simulink model "Tractor_HIT_Discrete"  (R2024a)
settings: Solver=ode1  StartTime=0.0  StopTime=60  FixedStep=0.001  RelTol=1e-3
values from neighbouring files (symbols this model uses):
  ANRtarget = 1.05    [Engine1204.sldd]    (also in Engine1204_init_r1.m; Engine2004.sldd; Engine2004_init.m; Engine3204.sldd)
  BackPrs = 3.0 4.2 5.5 7.0 8.5 10.0 11.5 12.5    [Engine1204.sldd]    (also in Engine1204_init_r1.m = [3.0, 4.2, 5.5, 7.0, 8.5, 10.0, 11.5, 12.5]; Engine2004.sldd = 3.0 4.2 5.5 7.0 8.5 10.0 11.5 12.5 13.5 14.5 15.0 15.5 16.0 ; Engine2004_init.m = [3.0,4.2,5.5,7.0,8.5,10.0,11.5,12.5,13.5,14.5,15.0,15.5,16.0; Engine3204.sldd = 3.0 4.5 6.0 7.5 9.0 10.5 12.0 13.0 13.8 14.4 14.8 15.2 15.6 )
  BackPrs_x = 50.0 100.0 150.0 200.0 250.0 300.0 350.0 400.0    [Engine1204.sldd]    (also in Engine1204_init_r1.m = [50:50:400]; Engine2004.sldd = 50.0 100.0 150.0 200.0 250.0 300.0 350.0 400.0 450.0 500.0 5; Engine2004_init.m = [50:50:800]; Engine3204.sldd = 100.0 200.0 300.0 400.0 500.0 600.0 700.0 800.0 900.0 1000.0)
  Bf = 0.38    [Engine1204.sldd]    (also in Engine2004.sldd; Engine3204.sldd)
  Br = 0.47    [Engine1204.sldd]    (also in Engine2004.sldd; Engine3204.sldd)
  BSFC = 320.0 285.0 275.0 280.0 290.0 300.0 310.0 260.0 225.0 215.0 220.0 228.0 240.0 250.0 235.0 208.0 202.0 205.0 212.0 222.0 232.0 230.0 205.0 200.0 204.0 210.0 220.0 230.0 232.0 207.0 203.0 206.0 213.0 224.0 235.0    [Engine1204.sldd]    (also in Engine1204_init_r1.m = [320,285,275,280,290,300,310; Engine2004.sldd = 315.0 280.0 270.0 275.0 285.0 295.0 305.0 255.0 220.0 210.0 ; Engine2004_init.m = [315,280,270,275,285,295,305; Engine3204.sldd = 310.0 275.0 265.0 270.0 280.0 290.0 300.0 250.0 215.0 205.0 )
  BSFC_x = 700.0 1200.0 1400.0 1600.0 1800.0 2000.0 2200.0    [Engine1204.sldd]    (also in Engine1204_init_r1.m = [700,1200,1400,1600,1800,2000,2200]; Engine2004.sldd = 800.0 1200.0 1400.0 1600.0 1800.0 2000.0 2200.0; Engine2004_init.m = [800,1200,1400,1600,1800,2000,2200]; Engine3204.sldd = 800.0 1000.0 1200.0 1400.0 1600.0 1800.0 2100.0)
  BSFC_y = 12.0 24.0 36.0 48.0 54.0    [Engine1204.sldd]    (also in Engine1204_init_r1.m = [12,24,36,48,54]; Engine2004.sldd = 20.0 40.0 60.0 80.0 100.0; Engine2004_init.m = [20,40,60,80,100]; Engine3204.sldd = 30.0 60.0 90.0 120.0 150.0)
  CO = 2.4 1.7 1.5 1.6 1.8 2.1 2.7 1.1 0.72 0.65 0.68 0.78 0.92 1.3 0.7 0.55 0.5 0.53 0.6 0.72 0.95 1.2 0.9 0.85 0.88 0.96 1.1 1.45 3.2 2.3 2.1 2.25 2.5 2.85 3.8    [Engine1204.sldd]    (also in Engine1204_init_r1.m = [; Engine2004.sldd = 2.3 1.63 1.44 1.54 1.73 2.02 2.56 1.05 0.68 0.61 0.64 0.74 0; Engine2004_init.m = [; Engine3204.sldd = 2.2 1.56 1.38 1.48 1.66 1.94 2.46 1.0 0.65 0.58 0.61 0.7 0.8)
  CO_x = 700.0 1200.0 1400.0 1600.0 1800.0 2000.0 2200.0    [Engine1204.sldd]    (also in Engine1204_init_r1.m = [700,1200,1400,1600,1800,2000,2200]; Engine2004.sldd = 800.0 1200.0 1400.0 1600.0 1800.0 2000.0 2200.0; Engine2004_init.m = [800,1200,1400,1600,1800,2000,2200]; Engine3204.sldd = 800.0 1000.0 1200.0 1400.0 1600.0 1800.0 2100.0)
  CO_y = 12.0 24.0 36.0 48.0 54.0    [Engine1204.sldd]    (also in Engine1204_init_r1.m = [12,24,36,48,54]; Engine2004.sldd = 20.0 40.0 60.0 80.0 100.0; Engine2004_init.m = [20,40,60,80,100]; Engine3204.sldd = 30.0 60.0 90.0 120.0 150.0)
  Df = 1.4    [Engine1204.sldd]    (also in Engine2004.sldd; Engine3204.sldd)
  dfmax = 0.1    [Engine1204.sldd]    (also in Engine2004.sldd; Engine3204.sldd)
  dfmin = 0.035    [Engine1204.sldd]    (also in Engine2004.sldd; Engine3204.sldd)
  DOCdPrs = 0.2 0.5 0.8 1.1 1.2    [Engine1204.sldd]    (also in Engine1204_init_r1.m = [0.2  0.5  0.8  1.1  1.2]; Engine2004.sldd = 0.25 0.55 0.85 1.15 1.3; Engine2004_init.m = [0.25,0.55,0.85,1.15,1.30]; Engine3204.sldd = 0.25 0.55 0.85 1.15 1.3 1.45)
  DOCdPrs_x = 50.0 150.0 250.0 350.0 400.0    [Engine1204.sldd]    (also in Engine1204_init_r1.m = [50  150  250  350  400]; Engine2004.sldd = 100.0 250.0 400.0 600.0 800.0; Engine2004_init.m = [100 250 400 600 800]; Engine3204.sldd = 100.0 250.0 400.0 600.0 800.0 1200.0)
  DPFdPrs = 0.3 0.5 0.7 0.9 0.6 1.0 1.4 1.8 0.9 1.5 2.1 2.6 1.2 2.0 2.7 2.8    [Engine1204.sldd]    (also in Engine1204_init_r1.m = [0.3  0.5  0.7  0.9; Engine2004.sldd = 0.35 0.6 0.85 1.1 0.7 1.15 1.6 2.0 1.05 1.7 2.3 2.5 1.4 2.2 ; Engine2004_init.m = [0.35,0.60,0.85,1.10; Engine3204.sldd = 0.35 0.7 1.05 1.4 1.7 2.0 2.2 2.4 2.55 2.65 2.7 2.75 0.6 1.1)
  DPFdPrs_x = 100.0 200.0 300.0 400.0    [Engine1204.sldd]    (also in Engine1204_init_r1.m = [100: 100 : 400]; Engine2004.sldd = 100.0 300.0 500.0 700.0; Engine2004_init.m = [100:200:700]; Engine3204.sldd = 100.0 200.0 300.0 400.0 500.0 600.0 700.0 800.0 900.0 1000.0)
  DPFdPrs_y = 0.0 6.0 12.0 20.0    [Engine1204.sldd]    (also in Engine1204_init_r1.m = [0 6 12 20 ]; Engine2004.sldd = 0.0 8.0 16.0 24.0; Engine2004_init.m = [0 8 16 24]; Engine3204.sldd = 0.0 10.0 20.0 30.0)
  DPFSootBurn = 0.0 0.0 0.0 0.0 0.0 0.2 0.4 0.6 0.8 1.0 1.2 2.4 3.6 4.8 6.0 6.0 12.0 18.0 24.0 30.0 12.0 24.0 36.0 48.0 60.0 20.0 40.0 60.0 80.0 100.0 22.0 44.0 66.0 88.0 110.0    [Engine1204.sldd]    (also in Engine1204_init_r1.m = [0,0,0,0,0; Engine2004.sldd = 0.0 0.0 0.0 0.0 0.0 0.5 1.0 1.5 2.0 2.5 3.0 6.0 9.0 12.0 15.; Engine2004_init.m = [0,0,0,0,0; Engine3204.sldd = 0.0 0.0 0.0 0.0 0.0 0.5 1.0 1.5 2.0 2.5 3.0 6.0 9.0 12.0 15.)
  DPFSootBurn_x = 100.0 200.0 300.0 400.0 500.0    [Engine1204.sldd]    (also in Engine1204_init_r1.m = [100,200,300,400,500]; Engine2004.sldd = 200.0 300.0 400.0 500.0 650.0; Engine2004_init.m = [200,300,400,500,650]; Engine3204.sldd = 200.0 300.0 400.0 500.0 650.0)
  DPFSootBurn_y = 400.0 450.0 500.0 550.0 600.0 650.0 680.0    [Engine1204.sldd]    (also in Engine1204_init_r1.m = [400,450,500,550,600,650,680]; Engine2004.sldd; Engine2004_init.m = [400,450,500,550,600,650,680]; Engine3204.sldd)
  Dr = 1.8    [Engine1204.sldd]    (also in Engine2004.sldd; Engine3204.sldd)
  drmax = 0.12    [Engine1204.sldd]    (also in Engine2004.sldd; Engine3204.sldd)
  drmin = 0.04    [Engine1204.sldd]    (also in Engine2004.sldd; Engine3204.sldd)
  EGRKi = 0.03    [Engine1204.sldd]    (also in Engine1204_init_r1.m; Engine2004.sldd; Engine2004_init.m; Engine3204.sldd)
  EGRKp = 3.5999999999999996    [Engine1204.sldd]    (also in Engine1204_init_r1.m = 3.6; Engine2004.sldd; Engine2004_init.m = 3.6; Engine3204.sldd)
  EGRMax = 1.0    [Engine1204.sldd]    (also in Engine1204_init_r1.m = 1; Engine2004.sldd; Engine2004_init.m = 1; Engine3204.sldd)
  EGRMin = 0.0    [Engine1204.sldd]    (also in Engine1204_init_r1.m = 0; Engine2004.sldd; Engine2004_init.m = 0; Engine3204.sldd)
  EGRRatio = 0.0 0.0 0.0 0.0 0.0 0.0 0.0 0.0 0.04 0.03 0.03 0.02 0.02 0.01 0.0 0.08 0.07 0.06 0.05 0.04 0.03 0.0 0.13 0.12 0.11 0.1 0.09 0.08 0.0 0.18 0.17 0.16 0.15 0.14 0.13 0.0 0.22 0.21 0.2 0.19 0.18 0.17    [Engine1204.sldd]    (also in Engine1204_init_r1.m = [; Engine2004.sldd; Engine2004_init.m = [; Engine3204.sldd)
  EGRRatio_x = 700.0 1200.0 1400.0 1600.0 1800.0 2000.0 2200.0    [Engine1204.sldd]    (also in Engine1204_init_r1.m = [700,1200,1400,1600,1800,2000,2200]; Engine2004.sldd = 800.0 1200.0 1400.0 1600.0 1800.0 2000.0 2200.0; Engine2004_init.m = [800,1200,1400,1600,1800,2000,2200]; Engine3204.sldd = 800.0 1000.0 1200.0 1400.0 1600.0 1800.0 2100.0)
  EGRRatio_y = 0.0 20.0 40.0 60.0 80.0 100.0    [Engine1204.sldd]    (also in Engine1204_init_r1.m = [0,20,40,60,80,100]; Engine2004.sldd; Engine2004_init.m = [0,20,40,60,80,100]; Engine3204.sldd)
  EGRTgt = 0.25 0.22 0.2 0.18 0.16 0.12 0.1 0.2 0.18 0.15 0.14 0.12 0.1 0.08 0.12 0.13 0.1 0.09 0.08 0.06 0.04 0.08 0.09 0.07 0.06 0.05 0.03 0.02 0.05 0.06 0.04 0.03 0.02 0.01 0.0    [Engine1204.sldd]    (also in Engine1204_init_r1.m = [0.25,0.22,0.20,0.18,0.16,0.12,0.10; Engine2004.sldd = 0.24 0.21 0.19 0.17 0.15 0.11 0.09 0.19 0.17 0.14 0.13 0.11 ; Engine2004_init.m = [0.24,0.21,0.19,0.17,0.15,0.11,0.09; Engine3204.sldd = 0.23 0.2 0.18 0.16 0.14 0.1 0.08 0.18 0.16 0.13 0.12 0.1 0.0)
  EGRTgt_x = 700.0 1200.0 1400.0 1600.0 1800.0 2000.0 2200.0    [Engine1204.sldd]    (also in Engine1204_init_r1.m = [700,1200,1400,1600,1800,2000,2200]; Engine2004.sldd = 800.0 1200.0 1400.0 1600.0 1800.0 2000.0 2200.0; Engine2004_init.m = [800,1200,1400,1600,1800,2000,2200]; Engine3204.sldd = 800.0 1000.0 1200.0 1400.0 1600.0 1800.0 2100.0)
  EGRTgt_y = 12.0 24.0 36.0 48.0 54.0    [Engine1204.sldd]    (also in Engine1204_init_r1.m = [12,24,36,48,54]; Engine2004.sldd = 20.0 40.0 60.0 80.0 100.0; Engine2004_init.m = [20,40,60,80,100]; Engine3204.sldd = 30.0 60.0 90.0 120.0 150.0)
  EGT = 197.0 257.0 287.0 297.0 287.0 267.0 247.0 267.0 357.0 397.0 407.0 392.0 367.0 347.0 337.0 437.0 472.0 482.0 462.0 437.0 407.0 367.0 477.0 502.0 512.0 492.0 467.0 437.0 377.0 487.0 510.0 520.0 500.0 477.0 447.0    [Engine1204.sldd]    (also in Engine1204_init_r1.m = [470,530,560,570,560,540,520; Engine2004.sldd = 187.0 247.0 277.0 287.0 277.0 257.0 237.0 257.0 347.0 387.0 ; Engine2004_init.m = [460,520,550,560,550,530,510; Engine3204.sldd = 307.0 327.0 338.0 327.0 307.0 277.0 237.0 322.0 337.0 332.0 )
  EGT_x = 700.0 1200.0 1400.0 1600.0 1800.0 2000.0 2200.0    [Engine1204.sldd]    (also in Engine1204_init_r1.m = [700,1200,1400,1600,1800,2000,2200]; Engine2004.sldd = 800.0 1200.0 1400.0 1600.0 1800.0 2000.0 2200.0; Engine2004_init.m = [800,1200,1400,1600,1800,2000,2200]; Engine3204.sldd = 800.0 1000.0 1200.0 1400.0 1600.0 1800.0 2100.0)
  EGT_y = 12.0 24.0 36.0 48.0 54.0    [Engine1204.sldd]    (also in Engine1204_init_r1.m = [12,24,36,48,54]; Engine2004.sldd = 20.0 40.0 60.0 80.0 100.0; Engine2004_init.m = [20,40,60,80,100]; Engine3204.sldd = 30.0 60.0 90.0 120.0 150.0)
  EngCsup = 0.35594 0.35501499999999997 0.353535 0.35242500000000004 0.351685 0.35150000000000003 0.35187 0.352795 0.35446 0.356865    [Engine1204.sldd]    (also in Engine2004.sldd; Engine3204.sldd)
  EngineSpdTgt = 700.0 850.0 1000.0 1150.0 1300.0 1450.0 1600.0 1750.0 1900.0 2050.0 2200.0    [Engine1204.sldd]    (also in Engine1204_init_r1.m = [700:150:2200]; Engine2004.sldd; Engine2004_init.m = [700:150:2200]; Engine3204.sldd = 800.0 930.0 1060.0 1190.0 1320.0 1450.0 1580.0 1710.0 1840.0)
  EngineSpdTgt_x = 0.0 10.0 20.0 30.0 40.0 50.0 60.0 70.0 80.0 90.0 100.0    [Engine1204.sldd]    (also in Engine1204_init_r1.m = [0:10:100]; Engine2004.sldd; Engine2004_init.m = [0:10:100]; Engine3204.sldd)
  EngineTrq = 70.0 110.0 130.0 125.0 115.0 100.0 85.0 180.0 280.0 320.0 310.0 285.0 250.0 220.0 260.0 370.0 410.0 395.0 365.0 320.0 280.0 300.0 420.0 450.0 435.0 400.0 350.0 300.0 310.0 435.0 460.0 445.0 410.0 355.0 305.0    [Engine1204.sldd]    (also in Engine1204_init_r1.m = [70,110,130,125,115,100,85; Engine2004.sldd = 130.0 200.0 240.0 230.0 210.0 180.0 150.0 320.0 480.0 550.0 ; Engine2004_init.m = [130,200,240,230,210,180,150; Engine3204.sldd = 210.0 320.0 380.0 360.0 330.0 290.0 240.0 510.0 760.0 870.0 )
  EngineTrq_x = 700.0 1200.0 1400.0 1600.0 1800.0 2000.0 2200.0    [Engine1204.sldd]    (also in Engine1204_init_r1.m = [700,1200,1400,1600,1800,2000,2200]; Engine2004.sldd = 800.0 1200.0 1400.0 1600.0 1800.0 2000.0 2200.0; Engine2004_init.m = [800,1200,1400,1600,1800,2000,2200]; Engine3204.sldd = 800.0 1000.0 1200.0 1400.0 1600.0 1800.0 2100.0)
  EngineTrq_y = 12.0 24.0 36.0 48.0 54.0    [Engine1204.sldd]    (also in Engine1204_init_r1.m = [12,24,36,48,54]; Engine2004.sldd = 20.0 40.0 60.0 80.0 100.0; Engine2004_init.m = [20,40,60,80,100]; Engine3204.sldd = 30.0 60.0 90.0 120.0 150.0)
  EngSpd = 800.0 1000.0 1200.0 1400.0 1600.0 1800.0 2000.0 2200.0 2400.0 2600.0    [Engine1204.sldd]    (also in Engine2004.sldd; Engine3204.sldd)
  EngTrq = 667.0 700.0 768.0 830.0 885.0 860.0 789.0 690.0 542.0 352.0    [Engine1204.sldd]    (also in Engine2004.sldd; Engine3204.sldd)
  etaCO = 0.0 0.0 0.0 0.0 0.6 0.45 0.3 0.15 0.92 0.85 0.75 0.6 0.98 0.95 0.9 0.82 0.99 0.97 0.94 0.88    [Engine1204.sldd]    (also in Engine1204_init_r1.m = [0.00	0.00	0.00	0.00; Engine2004.sldd; Engine2004_init.m = [0.00	0.00	0.00	0.00; Engine3204.sldd)
  etaCO_x = 10000.0 25000.0 40000.0 60000.0    [Engine1204.sldd]    (also in Engine1204_init_r1.m = [10000  25000  40000  60000]; Engine2004.sldd; Engine2004_init.m = [10000 25000 40000 60000]; Engine3204.sldd)
  etaCO_y = 120.0 200.0 280.0 360.0 450.0    [Engine1204.sldd]    (also in Engine1204_init_r1.m = [120, 200, 280, 360, 450]; Engine2004.sldd; Engine2004_init.m = [120,200,280,360,450]; Engine3204.sldd)
  etaHC = 0.0 0.0 0.0 0.0 0.5 0.35 0.2 0.1 0.88 0.8 0.68 0.5 0.96 0.92 0.86 0.75 0.98 0.95 0.91 0.83    [Engine1204.sldd]    (also in Engine1204_init_r1.m = [0.00	0.00	0.00	0.00; Engine2004.sldd; Engine2004_init.m = [0.00	0.00	0.00	0.00; Engine3204.sldd)
  etaHC_x = 10000.0 25000.0 40000.0 60000.0    [Engine1204.sldd]    (also in Engine1204_init_r1.m = [10000  25000  40000  60000]; Engine2004.sldd; Engine2004_init.m = [10000 25000 40000 60000]; Engine3204.sldd)
  etaHC_y = 120.0 200.0 280.0 360.0 450.0    [Engine1204.sldd]    (also in Engine1204_init_r1.m = [120, 200, 280, 360, 450]; Engine2004.sldd; Engine2004_init.m = [120,200,280,360,450]; Engine3204.sldd)
  etaNO2 = 0.0 0.0 0.0 0.0 0.2 0.15 0.1 0.05 0.4 0.33 0.25 0.18 0.55 0.48 0.4 0.3 0.6 0.53 0.45 0.35    [Engine1204.sldd]    (also in Engine1204_init_r1.m = [0.00	0.00	0.00	0.00; Engine2004.sldd; Engine2004_init.m = [0.00	0.00	0.00	0.00; Engine3204.sldd)
  etaNO2_x = 10000.0 25000.0 40000.0 60000.0    [Engine1204.sldd]    (also in Engine1204_init_r1.m = [10000  25000  40000  60000]; Engine2004.sldd; Engine2004_init.m = [10000 25000 40000 60000]; Engine3204.sldd)
  etaNO2_y = 120.0 200.0 280.0 360.0 450.0    [Engine1204.sldd]    (also in Engine1204_init_r1.m = [120, 200, 280, 360, 450]; Engine2004.sldd; Engine2004_init.m = [120,200,280,360,450]; Engine3204.sldd)
  etaPM = 0.995 0.992 0.988 0.98 0.996 0.994 0.99 0.985 0.997 0.995 0.992 0.988    [Engine1204.sldd]    (also in Engine1204_init_r1.m = [0.995  0.992  0.988  0.980; Engine2004.sldd; Engine2004_init.m = [0.995  0.992  0.988  0.980; Engine3204.sldd)
  etaPM_x = 10000.0 25000.0 40000.0 60000.0    [Engine1204.sldd]    (also in Engine1204_init_r1.m = [10000  25000  40000  60000]; Engine2004.sldd; Engine2004_init.m = [10000 25000 40000 60000]; Engine3204.sldd)
  etaPM_y = 150.0 300.0 450.0    [Engine1204.sldd]    (also in Engine1204_init_r1.m = [150, 300, 450]; Engine2004.sldd; Engine2004_init.m = [150,300,450]; Engine3204.sldd)
  FuelCyleMax = 40.0 45.0 50.0 52.0 54.0 50.0 60.0 65.0 66.0 68.0 52.0 64.0 66.0 67.0 68.0 50.0 62.0 64.0 65.0 66.0 48.0 58.0 60.0 61.0 62.0 42.0 50.0 52.0 53.0 54.0 38.0 44.0 46.0 47.0 48.0    [Engine1204.sldd]    (also in Engine1204_init_r1.m = [40,45,50,52,54; Engine2004.sldd = 65.0 75.0 82.0 88.0 92.0 75.0 88.0 94.0 98.0 102.0 78.0 92.0; Engine2004_init.m = [65,75,82,88,92; Engine3204.sldd = 95.0 110.0 125.0 140.0 155.0 110.0 130.0 145.0 160.0 175.0 1)
  FuelCyleMax_x = 80.0 140.0 200.0 260.0 320.0    [Engine1204.sldd]    (also in Engine1204_init_r1.m = [80,140,200,260,320]; Engine2004.sldd = 150.0 300.0 450.0 600.0 750.0; Engine2004_init.m = [150,300,450,600,750]; Engine3204.sldd = 250.0 500.0 750.0 1000.0 1300.0)
  FuelCyleMax_y = 700.0 1200.0 1400.0 1600.0 1800.0 2000.0 2200.0    [Engine1204.sldd]    (also in Engine1204_init_r1.m = [700,1200,1400,1600,1800,2000,2200]; Engine2004.sldd = 800.0 1200.0 1400.0 1600.0 1800.0 2000.0 2200.0; Engine2004_init.m = [800,1200,1400,1600,1800,2000,2200]; Engine3204.sldd = 800.0 1000.0 1200.0 1400.0 1600.0 1800.0 2100.0)
  FuelCyleMaxSw = 0.0    [Engine1204.sldd]    (also in Engine1204_init_r1.m = 0; Engine2004.sldd; Engine2004_init.m = 0; Engine3204.sldd)
  FuelCyleMin = 10.0    [Engine1204.sldd]    (also in Engine1204_init_r1.m = 10; Engine2004.sldd = 12.0; Engine2004_init.m = 12; Engine3204.sldd = 15.0)
  FuelKd = 0.0    [Engine1204.sldd]    (also in Engine1204_init_r1.m = 0; Engine2004.sldd; Engine2004_init.m = 0; Engine3204.sldd)
  FuelKi = 0.0162    [Engine1204.sldd]    (also in Engine1204_init_r1.m; Engine2004.sldd = 0.0198; Engine2004_init.m = 0.0198; Engine3204.sldd = 0.025199999999999997)
  FuelKp = 0.054    [Engine1204.sldd]    (also in Engine1204_init_r1.m; Engine2004.sldd = 0.066; Engine2004_init.m = 0.066; Engine3204.sldd = 0.083999999999999991)
  g = 9.81    [Engine1204.sldd]    (also in Engine2004.sldd; Engine3204.sldd)
  GearA = -2.9 0.0 6.0 2.5 1.0    [Engine1204.sldd]    (also in Engine2004.sldd; Engine3204.sldd)
  GearAC = -1.0 0.0 1.0 2.0 3.0    [Engine1204.sldd]    (also in Engine2004.sldd; Engine3204.sldd)
  GearFront = 17.574    [Engine1204.sldd]    (also in Engine2004.sldd; Engine3204.sldd)
  GearM = 2.33 1.75 1.4 1.0    [Engine1204.sldd]    (also in Engine2004.sldd; Engine3204.sldd)
  GearMC = 1.0 2.0 3.0 4.0    [Engine1204.sldd]    (also in Engine2004.sldd; Engine3204.sldd)
  GearRef = 14.6    [Engine1204.sldd]    (also in Engine2004.sldd; Engine3204.sldd)
  HC = 0.85 0.6 0.52 0.55 0.62 0.7 0.9 0.4 0.22 0.2 0.21 0.26 0.32 0.48 0.25 0.18 0.17 0.18 0.21 0.26 0.36 0.32 0.24 0.23 0.25 0.28 0.33 0.42 0.55 0.42 0.4 0.43 0.48 0.54 0.68    [Engine1204.sldd]    (also in Engine1204_init_r1.m = [; Engine2004.sldd = 0.82 0.58 0.5 0.53 0.6 0.68 0.87 0.38 0.21 0.19 0.2 0.24 0.3; Engine2004_init.m = [; Engine3204.sldd = 0.8 0.56 0.48 0.51 0.58 0.66 0.84 0.37 0.2 0.18 0.19 0.23 0.)
  HC_x = 700.0 1200.0 1400.0 1600.0 1800.0 2000.0 2200.0    [Engine1204.sldd]    (also in Engine1204_init_r1.m = [700,1200,1400,1600,1800,2000,2200]; Engine2004.sldd = 800.0 1200.0 1400.0 1600.0 1800.0 2000.0 2200.0; Engine2004_init.m = [800,1200,1400,1600,1800,2000,2200]; Engine3204.sldd = 800.0 1000.0 1200.0 1400.0 1600.0 1800.0 2100.0)
  HC_y = 12.0 24.0 36.0 48.0 54.0    [Engine1204.sldd]    (also in Engine1204_init_r1.m = [12,24,36,48,54]; Engine2004.sldd = 20.0 40.0 60.0 80.0 100.0; Engine2004_init.m = [20,40,60,80,100]; Engine3204.sldd = 30.0 60.0 90.0 120.0 150.0)
  hf = 0.35    [Engine1204.sldd]    (also in Engine2004.sldd; Engine3204.sldd)
  hr = 0.4    [Engine1204.sldd]    (also in Engine2004.sldd; Engine3204.sldd)
  IdleEngSpd = 700.0    [Engine1204.sldd]    (also in Engine2004.sldd; Engine3204.sldd)
  IdleThrottle = 0.3    [Engine1204.sldd]    (also in Engine2004.sldd; Engine3204.sldd)
  Inertia = 0.9    [Engine1204.sldd]    (also in Engine1204_init_r1.m; Engine2004.sldd = 1.4; Engine2004_init.m = 1.4; Engine3204.sldd = 2.0)
  Intake = 80.0 140.0 160.0 180.0 190.0 195.0 200.0 130.0 210.0 240.0 260.0 270.0 275.0 280.0 170.0 270.0 310.0 330.0 340.0 345.0 350.0 190.0 320.0 360.0 380.0 390.0 395.0 400.0 200.0 340.0 380.0 400.0 410.0 415.0 420.0    [Engine1204.sldd]    (also in Engine1204_init_r1.m = [80,140,160,180,190,195,200; Engine2004.sldd = 160.0 240.0 280.0 310.0 330.0 340.0 350.0 250.0 380.0 440.0 ; Engine2004_init.m = [160,240,280,310,330,340,350; Engine3204.sldd = 280.0 420.0 490.0 540.0 570.0 585.0 600.0 430.0 660.0 760.0 )
  Intake_x = 700.0 1200.0 1400.0 1600.0 1800.0 2000.0 2200.0    [Engine1204.sldd]    (also in Engine1204_init_r1.m = [700,1200,1400,1600,1800,2000,2200]; Engine2004.sldd = 800.0 1200.0 1400.0 1600.0 1800.0 2000.0 2200.0; Engine2004_init.m = [800,1200,1400,1600,1800,2000,2200]; Engine3204.sldd = 800.0 1000.0 1200.0 1400.0 1600.0 1800.0 2100.0)
  Intake_y = 12.0 24.0 36.0 48.0 54.0    [Engine1204.sldd]    (also in Engine1204_init_r1.m = [12,24,36,48,54]; Engine2004.sldd = 20.0 40.0 60.0 80.0 100.0; Engine2004_init.m = [20,40,60,80,100]; Engine3204.sldd = 30.0 60.0 90.0 120.0 150.0)
  IntakePrs = 1.0 1.1 1.22 1.35 1.48 1.6 1.7 1.0 1.12 1.24 1.37 1.5 1.62 1.72 1.0 1.13 1.25 1.38 1.51 1.63 1.73 1.0 1.14 1.26 1.39 1.52 1.64 1.74 1.0 1.15 1.27 1.4 1.53 1.65 1.75 1.0 1.16 1.28 1.41 1.54 1.66 1.76    [Engine1204.sldd]    (also in Engine1204_init_r1.m = [; Engine2004.sldd = 1.0 1.11 1.23 1.36 1.49 1.61 1.71 1.0 1.13 1.25 1.38 1.51 1.; Engine2004_init.m = [; Engine3204.sldd = 1.0 1.12 1.24 1.37 1.5 1.62 1.72 1.0 1.14 1.26 1.39 1.52 1.6)
  IntakePrs_x = 700.0 1200.0 1400.0 1600.0 1800.0 2000.0 2200.0    [Engine1204.sldd]    (also in Engine1204_init_r1.m = [700,1200,1400,1600,1800,2000,2200]; Engine2004.sldd = 800.0 1200.0 1400.0 1600.0 1800.0 2000.0 2200.0; Engine2004_init.m = [800,1200,1400,1600,1800,2000,2200]; Engine3204.sldd = 800.0 1000.0 1200.0 1400.0 1600.0 1800.0 2100.0)
  IntakePrs_y = 0.0 20.0 40.0 60.0 80.0 100.0    [Engine1204.sldd]    (also in Engine1204_init_r1.m = [0,20,40,60,80,100]; Engine2004.sldd; Engine2004_init.m = [0,20,40,60,80,100]; Engine3204.sldd)
  IntakePrsInit = 1.35    [Engine1204.sldd]    (also in Engine1204_init_r1.m; Engine2004.sldd; Engine2004_init.m; Engine3204.sldd)
  IntakeSw = 0    [Engine1204.sldd]    (also in Engine1204_init_r1.m = false; Engine2004.sldd; Engine2004_init.m = false; Engine3204.sldd)
  IntakeTC = 0.1    [Engine1204.sldd]    (also in Engine1204_init_r1.m; Engine2004.sldd; Engine2004_init.m; Engine3204.sldd)
  IntakeTemp = 25.0 28.0 30.0 32.0 34.0 36.0 38.0 25.0 38.0 40.0 42.0 44.0 46.0 48.0 25.0 48.0 50.0 52.0 54.0 56.0 58.0 25.0 58.0 60.0 62.0 64.0 66.0 68.0 25.0 66.0 68.0 70.0 72.0 74.0 76.0 25.0 72.0 74.0 76.0 78.0 80.0 82.0    [Engine1204.sldd]    (also in Engine1204_init_r1.m = [; Engine2004.sldd = 25.0 29.0 31.0 33.0 35.0 37.0 39.0 25.0 39.0 41.0 43.0 45.0 ; Engine2004_init.m = [; Engine3204.sldd = 25.0 30.0 32.0 34.0 36.0 38.0 40.0 25.0 40.0 42.0 44.0 46.0 )
  IntakeTemp_x = 700.0 1200.0 1400.0 1600.0 1800.0 2000.0 2200.0    [Engine1204.sldd]    (also in Engine1204_init_r1.m = [700,1200,1400,1600,1800,2000,2200]; Engine2004.sldd = 800.0 1200.0 1400.0 1600.0 1800.0 2000.0 2200.0; Engine2004_init.m = [800,1200,1400,1600,1800,2000,2200]; Engine3204.sldd = 800.0 1000.0 1200.0 1400.0 1600.0 1800.0 2100.0)
  IntakeTemp_y = 0.0 20.0 40.0 60.0 80.0 100.0    [Engine1204.sldd]    (also in Engine1204_init_r1.m = [0,20,40,60,80,100]; Engine2004.sldd; Engine2004_init.m = [0,20,40,60,80,100]; Engine3204.sldd)
  IntakeTempInit = 45.0    [Engine1204.sldd]    (also in Engine1204_init_r1.m = 45; Engine2004.sldd; Engine2004_init.m = 45; Engine3204.sldd)
  Jf = 180.0    [Engine1204.sldd]    (also in Engine2004.sldd; Engine3204.sldd)
  Jr = 450.0    [Engine1204.sldd]    (also in Engine2004.sldd; Engine3204.sldd)
  L = 2.75    [Engine1204.sldd]    (also in Engine2004.sldd; Engine3204.sldd)
  LiftTorque = 5000.0    [Engine1204.sldd]    (also in Engine2004.sldd; Engine3204.sldd)
  LoadTrqManu = 200.0    [Engine1204.sldd]    (also in Engine1204_init_r1.m = 200; Engine2004.sldd = 400.0; Engine2004_init.m = 400; Engine3204.sldd = 800.0)
  LoadTrqSW = 1    [Engine1204.sldd]    (also in Engine1204_init_r1.m = true; Engine2004.sldd; Engine2004_init.m = true; Engine3204.sldd = 0)
  M_I = 2500.0    [Engine1204.sldd]    (also in Engine2004.sldd; Engine3204.sldd)
  M_T = 6500.0    [Engine1204.sldd]    (also in Engine2004.sldd; Engine3204.sldd)
  MaxEngSpd = 2600.0    [Engine1204.sldd]    (also in Engine2004.sldd; Engine3204.sldd)
  NH3StoreMax = 0.0 1.2 2.0 2.4 2.2 1.7 1.1    [Engine1204.sldd]    (also in Engine1204_init_r1.m = [0  1.2  2.0  2.4  2.2  1.7  1.1]; Engine2004.sldd = 0.0 1.7 2.9 3.5 3.2 2.5 1.6; Engine2004_init.m = [0, 1.7, 2.9, 3.5, 3.2, 2.5, 1.6]; Engine3204.sldd = 0.0 2.2 3.8 4.5 4.2 3.3 2.1)
  NH3StoreMax_x = 180.0 220.0 260.0 300.0 340.0 380.0 420.0    [Engine1204.sldd]    (also in Engine1204_init_r1.m = [180  220  260  300  340  380  420]; Engine2004.sldd; Engine2004_init.m = [180 220 260 300 340 380 420]; Engine3204.sldd)
  NOx = 6.2 7.0 7.4 7.2 6.8 6.4 6.0 7.5 8.4 8.8 8.6 8.2 7.7 7.2 8.2 9.1 9.5 9.3 8.9 8.4 7.9 7.6 8.5 8.8 8.6 8.2 7.7 7.2 7.0 7.8 8.1 7.9 7.5 7.0 6.5    [Engine1204.sldd]    (also in Engine1204_init_r1.m = [6.2,7.0,7.4,7.2,6.8,6.4,6.0; Engine2004.sldd = 6.1 6.9 7.3 7.1 6.7 6.3 5.9 7.4 8.3 8.7 8.5 8.1 7.6 7.1 8.1 ; Engine2004_init.m = [6.1,6.9,7.3,7.1,6.7,6.3,5.9; Engine3204.sldd = 5.9 6.7 7.1 6.9 6.5 6.1 5.7 7.2 8.1 8.5 8.3 7.9 7.4 6.9 7.9 )
  NOx_x = 700.0 1200.0 1400.0 1600.0 1800.0 2000.0 2200.0    [Engine1204.sldd]    (also in Engine1204_init_r1.m = [700,1200,1400,1600,1800,2000,2200]; Engine2004.sldd = 800.0 1200.0 1400.0 1600.0 1800.0 2000.0 2200.0; Engine2004_init.m = [800,1200,1400,1600,1800,2000,2200]; Engine3204.sldd = 800.0 1000.0 1200.0 1400.0 1600.0 1800.0 2100.0)
  NOx_y = 12.0 24.0 36.0 48.0 54.0    [Engine1204.sldd]    (also in Engine1204_init_r1.m = [12,24,36,48,54]; Engine2004.sldd = 20.0 40.0 60.0 80.0 100.0; Engine2004_init.m = [20,40,60,80,100]; Engine3204.sldd = 30.0 60.0 90.0 120.0 150.0)
  NOxFac = 1.0 0.88 0.76 0.64 0.54 0.46 0.4    [Engine1204.sldd]    (also in Engine1204_init_r1.m = [1.00, 0.88, 0.76, 0.64, 0.54, 0.46, 0.40]; Engine2004.sldd; Engine2004_init.m = [1.00,0.88,0.76,0.64,0.54,0.46,0.40]; Engine3204.sldd)
  NOxFac_x = 0.0 0.05 0.1 0.15 0.19999999999999998 0.25 0.3    [Engine1204.sldd]    (also in Engine1204_init_r1.m = [0: 0.05 : 0.3]; Engine2004.sldd; Engine2004_init.m = [0:0.05:0.3]; Engine3204.sldd)
  NumCyl = 6.0    [Engine1204.sldd]    (also in Engine1204_init_r1.m = 6; Engine2004.sldd; Engine2004_init.m = 6; Engine3204.sldd)
  O2 = 16.5 16.0 15.8 15.5 15.2 14.8 14.5 13.0 12.2 11.8 11.5 11.2 10.8 10.5 9.5 8.6 8.0 7.7 7.4 7.0 6.7 7.0 6.2 5.6 5.3 5.0 4.7 4.4 6.0 5.3 4.8 4.5 4.2 4.0 3.8    [Engine1204.sldd]    (also in Engine1204_init_r1.m = [16.5,16.0,15.8,15.5,15.2,14.8,14.5; Engine2004.sldd = 16.3 15.8 15.6 15.3 15.0 14.6 14.3 12.8 12.0 11.6 11.3 11.0 ; Engine2004_init.m = [16.3,15.8,15.6,15.3,15.0,14.6,14.3; Engine3204.sldd = 16.0 15.5 15.3 15.0 14.7 14.3 14.0 12.5 11.7 11.3 11.0 10.7 )
  O2_x = 700.0 1200.0 1400.0 1600.0 1800.0 2000.0 2200.0    [Engine1204.sldd]    (also in Engine1204_init_r1.m = [700,1200,1400,1600,1800,2000,2200]; Engine2004.sldd = 800.0 1200.0 1400.0 1600.0 1800.0 2000.0 2200.0; Engine2004_init.m = [800,1200,1400,1600,1800,2000,2200]; Engine3204.sldd = 800.0 1000.0 1200.0 1400.0 1600.0 1800.0 2100.0)
  O2_y = 12.0 24.0 36.0 48.0 54.0    [Engine1204.sldd]    (also in Engine1204_init_r1.m = [12,24,36,48,54]; Engine2004.sldd = 20.0 40.0 60.0 80.0 100.0; Engine2004_init.m = [20,40,60,80,100]; Engine3204.sldd = 30.0 60.0 90.0 120.0 150.0)
  PM = 0.12 0.1 0.09 0.09 0.1 0.11 0.12 0.22 0.18 0.16 0.17 0.19 0.21 0.24 0.38 0.3 0.26 0.27 0.31 0.35 0.39 0.55 0.44 0.38 0.4 0.45 0.5 0.56 0.65 0.52 0.46 0.48 0.53 0.58 0.66    [Engine1204.sldd]    (also in Engine1204_init_r1.m = [0.12,0.10,0.09,0.09,0.10,0.11,0.12; Engine2004.sldd = 0.11 0.09 0.08 0.08 0.09 0.1 0.11 0.21 0.17 0.15 0.16 0.18 0; Engine2004_init.m = [0.11,0.09,0.08,0.08,0.09,0.10,0.11; Engine3204.sldd = 0.1 0.08 0.07 0.07 0.08 0.09 0.1 0.2 0.16 0.14 0.15 0.17 0.1)
  PM_x = 700.0 1200.0 1400.0 1600.0 1800.0 2000.0 2200.0    [Engine1204.sldd]    (also in Engine1204_init_r1.m = [700,1200,1400,1600,1800,2000,2200]; Engine2004.sldd = 800.0 1200.0 1400.0 1600.0 1800.0 2000.0 2200.0; Engine2004_init.m = [800,1200,1400,1600,1800,2000,2200]; Engine3204.sldd = 800.0 1000.0 1200.0 1400.0 1600.0 1800.0 2100.0)
  PM_y = 12.0 24.0 36.0 48.0 54.0    [Engine1204.sldd]    (also in Engine1204_init_r1.m = [12,24,36,48,54]; Engine2004.sldd = 20.0 40.0 60.0 80.0 100.0; Engine2004_init.m = [20,40,60,80,100]; Engine3204.sldd = 30.0 60.0 90.0 120.0 150.0)
  radps2rpm = 9.55    [Engine1204.sldd]    (also in Engine1204_init_r1.m; Engine2004.sldd; Engine2004_init.m; Engine3204.sldd)
  RailFuel = 400.0 600.0 700.0 700.0 650.0 600.0 550.0 600.0 800.0 900.0 900.0 850.0 800.0 750.0 700.0 1000.0 1100.0 1150.0 1100.0 1000.0 950.0 750.0 1200.0 1350.0 1350.0 1300.0 1200.0 1150.0 750.0 1300.0 1400.0 1450.0 1400.0 1300.0 1200.0    [Engine1204.sldd]    (also in Engine1204_init_r1.m = [400,600,700,700,650,600,550; Engine2004.sldd = 420.0 620.0 720.0 720.0 680.0 630.0 580.0 630.0 830.0 930.0 ; Engine2004_init.m = [420,620,720,720,680,630,580; Engine3204.sldd = 440.0 640.0 740.0 740.0 700.0 650.0 600.0 650.0 850.0 950.0 )
  RailFuel_x = 700.0 1200.0 1400.0 1600.0 1800.0 2000.0 2200.0    [Engine1204.sldd]    (also in Engine1204_init_r1.m = [700,1200,1400,1600,1800,2000,2200]; Engine2004.sldd = 800.0 1200.0 1400.0 1600.0 1800.0 2000.0 2200.0; Engine2004_init.m = [800,1200,1400,1600,1800,2000,2200]; Engine3204.sldd = 800.0 1000.0 1200.0 1400.0 1600.0 1800.0 2100.0)
  ... (+23 more)
undefined symbols (not defined in the file or in its folder): df, DiscIntNeverNeededParam, dr, MAP_AIR, MAP_EFF, MAP_EoCO, MAP_EoCO2, MAP_EoHC, MAP_EoNOx, MAP_EoPM, MAP_FUEL, MAP_FUELCMD, MAP_POWER, MAP_SPD, MAP_TEMPERATURE, NH3_MAX, R
libraries: simulink x9, slpidlib x5
(part 6 of 10)

== system Tractor_HIT_Discrete/WorkloadModel/Agricultural Implement/Chisel Plow4 ==
  note: 耕深
  note: 每齿犁宽
  note: 齿数
  VehSpd [m/s] : Inport
  LiftCmd [-] : Inport  Port=2
  Soil [-] : Inport  Port=3
  Action Port : ActionPort  ActionPortLabel=elseif( u1 == 4)
  4 : Subsystem
      mask DialogControl ParameterGroupVar Prompt: 参数
      mask Display: disp('Chisel Plow——凿形犁');
  Bus Creator1 : BusCreator  Inputs=4
  Constant : Constant  Value=0
  Constant1 : Constant  Value=0
  Constant2 : Constant
  Constant3 : Constant  Value=0.85
  Constant4 : Constant  Value=0.65
  Data Store Write : DataStoreWrite  DataStoreName=Width  IndexOptions=Index vector (dialog)  Indices=1  OutputSizes=1
  Data Store Write1 : DataStoreWrite  DataStoreName=PtoTrq  IndexOptions=Index vector (dialog)  Indices=1  OutputSizes=1
  Data Store Write2 : DataStoreWrite  DataStoreName=Draught  IndexOptions=Index vector (dialog)  Indices=1  OutputSizes=1
  Data Store Write3 : DataStoreWrite  DataStoreName=PwrPTO  IndexOptions=Index vector (dialog)  Indices=1  OutputSizes=1
  Data Store Write4 : DataStoreWrite  DataStoreName=PwrDraught  IndexOptions=Index vector (dialog)  Indices=1  OutputSizes=1
  Data Store Write5 : DataStoreWrite  DataStoreName=LiftTorque  IndexOptions=Index vector (dialog)  Indices=1  OutputSizes=1
  DepthCmd4[cm] : Constant  Value=5
  Gain : Gain  Gain=3.6
  Gain2 : Gain  Gain=0.001
  LiftTorque : Constant  Value=LiftTorque
  Multiport Switch : MultiPortSwitch  DataPortOrder=Zero-based contiguous  zeroidx=on  SaturateOnIntegerOverflow=off  InputSameDT=off
  Product : Product
  Switch : Switch  Criteria=u2 > Threshold  SaturateOnIntegerOverflow=off  InputSameDT=off
  Switch1 : Switch  Criteria=u2 > Threshold  SaturateOnIntegerOverflow=off  InputSameDT=off
  ToolsCmd4[-] : Constant  Value=6
  WidthCmd4[m] : Constant  Value=0.3
  Zero : Constant  Value=0  OutDataTypeStr=Inherit: Inherit via back propagation
  wires:
  Constant1/1 -> Switch1/3
  Constant/1 -> Switch/1
  4/1(Width[m]) -> Data Store Write/1
  Switch1/1 -> Data Store Write5/1
  LiftCmd [-]/1 -> Switch/2, Switch1/2
  Zero/1 -> Data Store Write3/1, Data Store Write1/1
  Switch/1 -> Product/1, Data Store Write2/1
  LiftTorque/1 -> Switch1/1
  Product/1 -> Gain2/1
  Gain2/1 -> Data Store Write4/1
  Gain/1 -> 4/1(Velocity)
  4/2(draft force) -> Switch/3
  [TillageCmd] -> 4/2(TIllageCmd)
  WidthCmd4[m]/1 -> Bus Creator1/3  "WidthCmd"
  ToolsCmd4[-]/1 -> Bus Creator1/2  "ToolsCmd"
  Bus Creator1/1 -> [TillageCmd]
  DepthCmd4[cm]/1 -> Bus Creator1/4  "DepthCmd"
  VehSpd [m/s]/1 -> Gain/1, Product/2
  Soil [-]/1 -> Multiport Switch/1
  Constant4/1 -> Multiport Switch/4
  Constant2/1 -> Multiport Switch/2
  Constant3/1 -> Multiport Switch/3
  Multiport Switch/1 -> Bus Creator1/1  "FiCmd"

== system Tractor_HIT_Discrete/WorkloadModel/Agricultural Implement/Cultivator0 ==
  note: 土壤参数
  note: 耕深
  note: 每齿犁宽
  note: 齿数
  VehSpd [m/s] : Inport
  LiftCmd [-] : Inport  Port=2
  Soil [-] : Inport  Port=3
  Action Port : ActionPort  ActionPortLabel=if(u1 == 0)
  Bus Creator1 : BusCreator  Inputs=4
  Constant : Constant  Value=0
  Constant1 : Constant  Value=0
  Constant2 : Constant
  Constant3 : Constant  Value=0.85
  Constant4 : Constant  Value=0.65
  Data Store Write : DataStoreWrite  DataStoreName=Width  IndexOptions=Index vector (dialog)  Indices=1  OutputSizes=1
  Data Store Write1 : DataStoreWrite  DataStoreName=PtoTrq  IndexOptions=Index vector (dialog)  Indices=1  OutputSizes=1
  Data Store Write2 : DataStoreWrite  DataStoreName=Draught  IndexOptions=Index vector (dialog)  Indices=1  OutputSizes=1
  Data Store Write3 : DataStoreWrite  DataStoreName=PwrPTO  IndexOptions=Index vector (dialog)  Indices=1  OutputSizes=1
  Data Store Write4 : DataStoreWrite  DataStoreName=PwrDraught  IndexOptions=Index vector (dialog)  Indices=1  OutputSizes=1
  Data Store Write5 : DataStoreWrite  DataStoreName=LiftTorque  IndexOptions=Index vector (dialog)  Indices=1  OutputSizes=1
  DepthCmd0[cm] : Constant  Value=5
  Gain : Gain  Gain=3.6
  Gain2 : Gain  Gain=0.001
  LiftTorque : Constant  Value=LiftTorque
  Multiport Switch : MultiPortSwitch  DataPortOrder=Zero-based contiguous  zeroidx=on  SaturateOnIntegerOverflow=off  InputSameDT=off
  Product : Product
  Switch : Switch  Criteria=u2 > Threshold  SaturateOnIntegerOverflow=off  InputSameDT=off
  Switch1 : Switch  Criteria=u2 > Threshold  SaturateOnIntegerOverflow=off  InputSameDT=off
  ToolsCmd0[-] : Constant  Value=6
  WidthCmd0[m] : Constant  Value=0.3
  Zero : Constant  Value=0  OutDataTypeStr=Inherit: Inherit via back propagation
  draught : Subsystem
      mask DialogControl ParameterGroupVar Prompt: 参数
      mask Display: disp('Field Cultivator for primary tillage——用于初耕的耕耘机');
  wires:
  Constant1/1 -> Switch1/3
  Constant/1 -> Switch/1
  draught/1(Width[m]) -> Data Store Write/1
  Switch1/1 -> Data Store Write5/1
  LiftCmd [-]/1 -> Switch/2, Switch1/2
  Zero/1 -> Data Store Write3/1, Data Store Write1/1
  Switch/1 -> Product/1, Data Store Write2/1
  LiftTorque/1 -> Switch1/1
  Product/1 -> Gain2/1
  Gain2/1 -> Data Store Write4/1
  Gain/1 -> draught/1(Velocity)
  draught/2(draft force) -> Switch/3
  [TillageCmd] -> draught/2(TIllageCmd)
  WidthCmd0[m]/1 -> Bus Creator1/3  "WidthCmd"
  ToolsCmd0[-]/1 -> Bus Creator1/2  "ToolsCmd"
  Bus Creator1/1 -> [TillageCmd]
  Multiport Switch/1 -> Bus Creator1/1  "FiCmd"
  DepthCmd0[cm]/1 -> Bus Creator1/4  "DepthCmd"
  VehSpd [m/s]/1 -> Gain/1, Product/2
  Constant2/1 -> Multiport Switch/2
  Soil [-]/1 -> Multiport Switch/1
  Constant3/1 -> Multiport Switch/3
  Constant4/1 -> Multiport Switch/4

== system Tractor_HIT_Discrete/WorkloadModel/Agricultural Implement/Fluctuation_Calc ==
  Soil[-] : Inport
  Scene[-] : Inport  Port=2
  Abs1 : Abs  SaturateOnIntegerOverflow=off
  Add : Sum
  Multiport Switch1 : MultiPortSwitch  DataPortOrder=Zero-based contiguous  zeroidx=on  SaturateOnIntegerOverflow=off  InputSameDT=off
  Random Number : RandomNumber  Mean=500  Variance=100  SampleTime=0.1
  Random Number1 : RandomNumber  Mean=100  Variance=100  SampleTime=0.1
  Random Number2 : RandomNumber  Mean=50  Variance=100  SampleTime=0.1
  Repeating Sequence Stair : simulink/Sources/Repeating Sequence Stair  OutValues=[3 1 4 2 1]*100  tsamp=0.01  OutMin=[]  OutMax=[]  OutDataTypeStr=double  OutputDataTypeScalingMode=double  OutDataType=fixdt(0,8)  ConRadixGroup=Best Precision: Vector-wise  OutScaling=2^-12
  Repeating Sequence Stair1 : simulink/Sources/Repeating Sequence Stair  OutValues=[3 1 4 2 1]*50  tsamp=0.01  OutMin=[]  OutMax=[]  OutDataTypeStr=double  OutputDataTypeScalingMode=double  OutDataType=fixdt(0,8)  ConRadixGroup=Best Precision: Vector-wise  OutScaling=2^-12
  Switch : Switch  Threshold=2  SaturateOnIntegerOverflow=off  InputSameDT=off
  Fluctuation[N] : Outport
  wires:
  Random Number/1 -> Multiport Switch1/2
  Random Number2/1 -> Multiport Switch1/4
  Random Number1/1 -> Multiport Switch1/3
  Multiport Switch1/1 -> Abs1/1
  Soil[-]/1 -> Multiport Switch1/1
  Scene[-]/1 -> Switch/2
  Abs1/1 -> Add/1
  Add/1 -> Fluctuation[N]/1
  Repeating Sequence Stair/1 -> Switch/1
  Repeating Sequence Stair1/1 -> Switch/3
  Switch/1 -> Add/2

== system Tractor_HIT_Discrete/WorkloadModel/Agricultural Implement/Moldboard Plow1 ==
  note: 耕深
  note: 每齿犁宽
  note: 齿数
  VehSpd [m/s] : Inport
  LiftCmd [-] : Inport  Port=2
  Soil [-] : Inport  Port=3
  Action Port : ActionPort  ActionPortLabel=elseif(u1 == 1)
  1 : Subsystem
      mask Display: disp('moldboard plow——铧式犁');
  Bus Creator1 : BusCreator  Inputs=4
  Constant : Constant  Value=0
  Constant1 : Constant  Value=0
  Constant2 : Constant
  Constant3 : Constant  Value=0.7
  Constant4 : Constant  Value=0.45
  Data Store Write : DataStoreWrite  DataStoreName=Width  IndexOptions=Index vector (dialog)  Indices=1  OutputSizes=1
  Data Store Write1 : DataStoreWrite  DataStoreName=PtoTrq  IndexOptions=Index vector (dialog)  Indices=1  OutputSizes=1
  Data Store Write2 : DataStoreWrite  DataStoreName=Draught  IndexOptions=Index vector (dialog)  Indices=1  OutputSizes=1
  Data Store Write3 : DataStoreWrite  DataStoreName=PwrPTO  IndexOptions=Index vector (dialog)  Indices=1  OutputSizes=1
  Data Store Write4 : DataStoreWrite  DataStoreName=PwrDraught  IndexOptions=Index vector (dialog)  Indices=1  OutputSizes=1
  Data Store Write5 : DataStoreWrite  DataStoreName=LiftTorque  IndexOptions=Index vector (dialog)  Indices=1  OutputSizes=1
  DepthCmd1[cm] : Constant  Value=25
  Gain : Gain  Gain=3.6
  Gain2 : Gain  Gain=0.001
  LiftTrq : Constant  Value=LiftTorque
  Multiport Switch : MultiPortSwitch  DataPortOrder=Zero-based contiguous  zeroidx=on  SaturateOnIntegerOverflow=off  InputSameDT=off
  Product : Product
  Switch : Switch  Criteria=u2 > Threshold  SaturateOnIntegerOverflow=off  InputSameDT=off
  Switch1 : Switch  Criteria=u2 > Threshold  SaturateOnIntegerOverflow=off  InputSameDT=off
  ToolsCmd1[-] : Constant  Value=4
  WidthCmd1[m] : Constant  Value=0.5
  Zero : Constant  Value=0  OutDataTypeStr=Inherit: Inherit via back propagation
  wires:
  Constant1/1 -> Switch1/3
  Constant/1 -> Switch/1
  1/1(Width[m]) -> Data Store Write/1
  Switch1/1 -> Data Store Write5/1
  LiftCmd [-]/1 -> Switch/2, Switch1/2
  Zero/1 -> Data Store Write3/1, Data Store Write1/1
  Switch/1 -> Product/1, Data Store Write2/1
  LiftTrq/1 -> Switch1/1
  Product/1 -> Gain2/1
  Gain2/1 -> Data Store Write4/1
  Gain/1 -> 1/1(Velocity)
  1/2(draft force) -> Switch/3
  [TillageCmd] -> 1/2(TillageCmd)
  WidthCmd1[m]/1 -> Bus Creator1/3  "WidthCmd"
  ToolsCmd1[-]/1 -> Bus Creator1/2  "ToolsCmd"
  Bus Creator1/1 -> [TillageCmd]
  DepthCmd1[cm]/1 -> Bus Creator1/4  "DepthCmd"
  VehSpd [m/s]/1 -> Gain/1, Product/2
  Constant4/1 -> Multiport Switch/4
  Constant2/1 -> Multiport Switch/2
  Constant3/1 -> Multiport Switch/3
  Multiport Switch/1 -> Bus Creator1/1  "FiCmd"
  Soil [-]/1 -> Multiport Switch/1

== system Tractor_HIT_Discrete/WorkloadModel/Agricultural Implement/PTO ==
  PTOSpdCmd [-] : Inport
  VehSpd [m/s] : Inport  Port=2
  Action Port : ActionPort  ActionPortLabel=elseif( u1==6)
  0 : Constant  Value=0  OutDataTypeStr=Inherit: Inherit via back propagation
  1 : Constant  Value=540  OutDataTypeStr=Inherit: Inherit via back propagation
  2 : Constant  Value=1000  OutDataTypeStr=Inherit: Inherit via back propagation
  Constant : Constant  Value=500
  Constant1 : Constant  Value=0
  Data Store Write : DataStoreWrite  DataStoreName=Width  IndexOptions=Index vector (dialog)  Indices=1  OutputSizes=1
  Data Store Write1 : DataStoreWrite  DataStoreName=PtoTrq  IndexOptions=Index vector (dialog)  Indices=1  OutputSizes=1
  Data Store Write2 : DataStoreWrite  DataStoreName=Draught  IndexOptions=Index vector (dialog)  Indices=1  OutputSizes=1
  Data Store Write3 : DataStoreWrite  DataStoreName=PwrPTO  IndexOptions=Index vector (dialog)  Indices=1  OutputSizes=1
  Data Store Write4 : DataStoreWrite  DataStoreName=PwrDraught  IndexOptions=Index vector (dialog)  Indices=1  OutputSizes=1
  Fcn : Fcn  Expr=0.9*u
  Gain2 : Gain  Gain=0.001
  Multiport Switch1 : MultiPortSwitch  DataPortOrder=Zero-based contiguous  Inputs=4  zeroidx=on  SaturateOnIntegerOverflow=off  InputSameDT=off
  Product : Product
  Product1 : Product
  PtoWidth : Constant  Value=2
  rpm2rad/s : Gain  Gain=1/9.55
  wires:
  1/1 -> Multiport Switch1/3
  Constant/1 -> Product/1
  Product/1 -> Multiport Switch1/5
  0/1 -> Multiport Switch1/2
  2/1 -> Multiport Switch1/4
  Multiport Switch1/1 -> rpm2rad/s/1, Fcn/1
  PTOSpdCmd [-]/1 -> Multiport Switch1/1
  Fcn/1 -> Data Store Write1/1, Product1/1
  Gain2/1 -> Data Store Write3/1
  rpm2rad/s/1 -> Product1/2
  Product1/1 -> Gain2/1
  PtoWidth/1 -> Data Store Write/1
  VehSpd [m/s]/1 -> Product/2
  Constant1/1 -> Data Store Write4/1, Data Store Write2/1

== system Tractor_HIT_Discrete/WorkloadModel/Agricultural Implement/Paddy Implement5 ==
  note: 耕深
  note: 每齿犁宽
  note: 齿数
  VehSpd [m/s] : Inport
  LiftCmd [-] : Inport  Port=2
  Soil [-] : Inport  Port=3
  Action Port : ActionPort  ActionPortLabel=elseif( u1 == 5)
  Constant : Constant  Value=0
  Constant1 : Constant  Value=0
  Constant2 : Constant  Value=4
  Constant3 : Constant  Value=3
  Constant4 : Constant  Value=2
  Data Store Write : DataStoreWrite  DataStoreName=Width  IndexOptions=Index vector (dialog)  Indices=1  OutputSizes=1
  Data Store Write1 : DataStoreWrite  DataStoreName=PtoTrq  IndexOptions=Index vector (dialog)  Indices=1  OutputSizes=1
  Data Store Write2 : DataStoreWrite  DataStoreName=Draught  IndexOptions=Index vector (dialog)  Indices=1  OutputSizes=1
  Data Store Write3 : DataStoreWrite  DataStoreName=PwrPTO  IndexOptions=Index vector (dialog)  Indices=1  OutputSizes=1
  Data Store Write4 : DataStoreWrite  DataStoreName=PwrDraught  IndexOptions=Index vector (dialog)  Indices=1  OutputSizes=1
  Data Store Write5 : DataStoreWrite  DataStoreName=LiftTorque  IndexOptions=Index vector (dialog)  Indices=1  OutputSizes=1
  DepthCmd5[cm] : Constant  Value=10
  Gain : Gain  Gain=100
  Gain2 : Gain  Gain=0.001
  LiftTorque : Constant  Value=LiftTorque
  Multiport Switch : MultiPortSwitch  DataPortOrder=Zero-based contiguous  zeroidx=on  SaturateOnIntegerOverflow=off  InputSameDT=off
  Product : Product
  Product1 : Product  Inputs=4
  Product2 : Product
  Switch : Switch  Criteria=u2 > Threshold  SaturateOnIntegerOverflow=off  InputSameDT=off
  Switch1 : Switch  Criteria=u2 > Threshold  SaturateOnIntegerOverflow=off  InputSameDT=off
  ToolsCmd5[-] : Constant  Value=5
  WidthCmd5[m] : Constant  Value=0.3
  Zero : Constant  Value=0  OutDataTypeStr=Inherit: Inherit via back propagation
  wires:
  Gain/1 -> Product1/3
  Multiport Switch/1 -> Product1/1
  DepthCmd5[cm]/1 -> Product1/2
  Product1/1 -> Switch/3
  WidthCmd5[m]/1 -> Product2/2  "WidthCmd"
  Product2/1 -> Data Store Write/1, Gain/1
  Constant/1 -> Switch/1
  Switch1/1 -> Data Store Write5/1
  VehSpd [m/s]/1 -> Product1/4, Product/2
  LiftCmd [-]/1 -> Switch1/2, Switch/2
  Switch/1 -> Data Store Write2/1, Product/1
  Zero/1 -> Data Store Write1/1, Data Store Write3/1
  Constant1/1 -> Switch1/3
  LiftTorque/1 -> Switch1/1
  Product/1 -> Gain2/1
  Gain2/1 -> Data Store Write4/1
  ToolsCmd5[-]/1 -> Product2/1  "ToolsCmd"
  Soil [-]/1 -> Multiport Switch/1
  Constant2/1 -> Multiport Switch/2
  Constant3/1 -> Multiport Switch/3
  Constant4/1 -> Multiport Switch/4

== system Tractor_HIT_Discrete/WorkloadModel/Agricultural Implement/Subsoiler3 ==
  note: 耕深
  note: 每齿犁宽
  note: 齿数
  VehSpd [m/s] : Inport
  LiftCmd [-] : Inport  Port=2
  Soil [-] : Inport  Port=3
  Action Port : ActionPort  ActionPortLabel=elseif( u1 == 3)
  3 : Subsystem
      mask DialogControl ParameterGroupVar Prompt: 参数
      mask Display: disp('Subsoiler——深松机');
  Bus Creator1 : BusCreator  Inputs=4
  Constant : Constant  Value=0
  Constant1 : Constant  Value=0
  Constant2 : Constant
  Constant3 : Constant  Value=0.7
  Constant4 : Constant  Value=0.45
  Data Store Write : DataStoreWrite  DataStoreName=Width  IndexOptions=Index vector (dialog)  Indices=1  OutputSizes=1
  Data Store Write1 : DataStoreWrite  DataStoreName=PtoTrq  IndexOptions=Index vector (dialog)  Indices=1  OutputSizes=1
  Data Store Write2 : DataStoreWrite  DataStoreName=Draught  IndexOptions=Index vector (dialog)  Indices=1  OutputSizes=1
  Data Store Write3 : DataStoreWrite  DataStoreName=PwrPTO  IndexOptions=Index vector (dialog)  Indices=1  OutputSizes=1
  Data Store Write4 : DataStoreWrite  DataStoreName=PwrDraught  IndexOptions=Index vector (dialog)  Indices=1  OutputSizes=1
  Data Store Write5 : DataStoreWrite  DataStoreName=LiftTorque  IndexOptions=Index vector (dialog)  Indices=1  OutputSizes=1
  DepthCmd3[cm] : Constant  Value=5
  Gain : Gain  Gain=3.6
  Gain2 : Gain  Gain=0.001
  LiftTorque : Constant  Value=LiftTorque
  Multiport Switch : MultiPortSwitch  DataPortOrder=Zero-based contiguous  zeroidx=on  SaturateOnIntegerOverflow=off  InputSameDT=off
  Product : Product
  Switch : Switch  Criteria=u2 > Threshold  SaturateOnIntegerOverflow=off  InputSameDT=off
  Switch1 : Switch  Criteria=u2 > Threshold  SaturateOnIntegerOverflow=off  InputSameDT=off
  ToolsCmd3[-] : Constant  Value=6
  WidthCmd3[m] : Constant  Value=0.3
  Zero : Constant  Value=0  OutDataTypeStr=Inherit: Inherit via back propagation
  wires:
  Constant1/1 -> Switch1/3
  Constant/1 -> Switch/1
  3/1(Width[m]) -> Data Store Write/1
  Switch1/1 -> Data Store Write5/1
  LiftCmd [-]/1 -> Switch/2, Switch1/2
  Zero/1 -> Data Store Write3/1, Data Store Write1/1
  Switch/1 -> Product/1, Data Store Write2/1
  LiftTorque/1 -> Switch1/1
  Product/1 -> Gain2/1
  Gain2/1 -> Data Store Write4/1
  Gain/1 -> 3/1(Velocity)
  3/2(draft force) -> Switch/3
  [TillageCmd] -> 3/2(TIllageCmd)
  WidthCmd3[m]/1 -> Bus Creator1/3  "WidthCmd"
  ToolsCmd3[-]/1 -> Bus Creator1/2  "ToolsCmd"
  Bus Creator1/1 -> [TillageCmd]
  DepthCmd3[cm]/1 -> Bus Creator1/4  "DepthCmd"
  VehSpd [m/s]/1 -> Gain/1, Product/2
  Constant3/1 -> Multiport Switch/3
  Constant2/1 -> Multiport Switch/2
  Multiport Switch/1 -> Bus Creator1/1  "FiCmd"
  Soil [-]/1 -> Multiport Switch/1
  Constant4/1 -> Multiport Switch/4

== system Tractor_HIT_Discrete/WorkloadModel/Agricultural Implement/Sweep Plow2 ==
  note: 耕深
  note: 每齿犁宽
  note: 齿数
  VehSpd [m/s] : Inport
  LiftCmd [-] : Inport  Port=2
  Soil [-] : Inport  Port=3
  Action Port : ActionPort  ActionPortLabel=elseif( u1 == 2)
  2 : Subsystem
      mask DialogControl ParameterGroupVar Prompt: 参数
      mask Display: disp('Sweep Plow for primary tillage——用于初耕的扫地犁');
  Bus Creator1 : BusCreator  Inputs=4
  Constant : Constant  Value=0
  Constant1 : Constant  Value=0
  Constant2 : Constant
  Constant3 : Constant  Value=0.85
  Constant4 : Constant  Value=0.65
  Data Store Write : DataStoreWrite  DataStoreName=Width  IndexOptions=Index vector (dialog)  Indices=1  OutputSizes=1
  Data Store Write1 : DataStoreWrite  DataStoreName=PtoTrq  IndexOptions=Index vector (dialog)  Indices=1  OutputSizes=1
  Data Store Write2 : DataStoreWrite  DataStoreName=Draught  IndexOptions=Index vector (dialog)  Indices=1  OutputSizes=1
  Data Store Write3 : DataStoreWrite  DataStoreName=PwrPTO  IndexOptions=Index vector (dialog)  Indices=1  OutputSizes=1
  Data Store Write4 : DataStoreWrite  DataStoreName=PwrDraught  IndexOptions=Index vector (dialog)  Indices=1  OutputSizes=1
  Data Store Write5 : DataStoreWrite  DataStoreName=LiftTorque  IndexOptions=Index vector (dialog)  Indices=1  OutputSizes=1
  DepthCmd2[cm] : Constant  Value=5
  Gain : Gain  Gain=3.6
  Gain2 : Gain  Gain=0.001
  LiftTorque : Constant  Value=LiftTorque
  Multiport Switch : MultiPortSwitch  DataPortOrder=Zero-based contiguous  zeroidx=on  SaturateOnIntegerOverflow=off  InputSameDT=off
  Product : Product
  Switch : Switch  Criteria=u2 > Threshold  SaturateOnIntegerOverflow=off  InputSameDT=off
  Switch1 : Switch  Criteria=u2 > Threshold  SaturateOnIntegerOverflow=off  InputSameDT=off
  ToolsCmd2[-] : Constant  Value=6
  WidthCmd2[m] : Constant  Value=0.3
  Zero : Constant  Value=0  OutDataTypeStr=Inherit: Inherit via back propagation
  wires:
  Constant1/1 -> Switch1/3
  Constant/1 -> Switch/1
  2/1(Width[m]) -> Data Store Write/1
  Switch1/1 -> Data Store Write5/1
  LiftCmd [-]/1 -> Switch/2, Switch1/2
  Zero/1 -> Data Store Write3/1, Data Store Write1/1
  Switch/1 -> Product/1, Data Store Write2/1
  LiftTorque/1 -> Switch1/1
  Product/1 -> Gain2/1
  Gain2/1 -> Data Store Write4/1
  Gain/1 -> 2/1(Velocity)
  2/2(draft force1) -> Switch/3
  [TillageCmd] -> 2/2(TIllageCmd)
  WidthCmd2[m]/1 -> Bus Creator1/3  "WidthCmd"
  ToolsCmd2[-]/1 -> Bus Creator1/2  "ToolsCmd"
  Bus Creator1/1 -> [TillageCmd]
  DepthCmd2[cm]/1 -> Bus Creator1/4  "DepthCmd"
  VehSpd [m/s]/1 -> Gain/1, Product/2
  Constant2/1 -> Multiport Switch/2
  Multiport Switch/1 -> Bus Creator1/1  "FiCmd"
  Soil [-]/1 -> Multiport Switch/1
  Constant3/1 -> Multiport Switch/3
  Constant4/1 -> Multiport Switch/4

== system Tractor_HIT_Discrete/WorkloadModel/Tires and Ground/Bn_Calc_single ==
  Fzf : Inport
  Fzr : Inport  Port=2
  Scene[-] : Inport  Port=3
  CI[kPa] : Inport  Port=4
  Demux : Demux  Outputs=2
  Mux : Mux  Inputs=2
  Mux1 : Mux  Inputs=2
  Subsystem2 : Subsystem
  Switch : Switch  Criteria=u2 ~= 0  SaturateOnIntegerOverflow=off  InputSameDT=off
  kPa2Pa : Gain  Gain=1000
  旱田 : Subsystem
  水田 : Subsystem
  Bn_f : Outport
  Bn_r : Outport  Port=2
  wires:
  CI[kPa]/1 -> kPa2Pa/1
  Scene[-]/1 -> Switch/2
  Switch/1 -> Demux/1
  Demux/1 -> Bn_f/1
  Demux/2 -> Bn_r/1
  Mux/1 -> Switch/1
  旱田/1(Bn_f) -> Mux/1
  旱田/2(Bn_r) -> Mux/2
  水田/1(Bn_f) -> Mux1/1
  水田/2(Bn_r) -> Mux1/2
  Mux1/1 -> Switch/3
  Subsystem2/2(Cn_r) -> 水田/2(Cn_r), 旱田/2(Cn_r)
  Subsystem2/1(Cn_f) -> 水田/1(Cn_f), 旱田/1(Cn_f)
  kPa2Pa/1 -> Subsystem2/1(CI[Pa])
  Fzf/1 -> Subsystem2/2(Fzf[N])
  Fzr/1 -> Subsystem2/3(Fzr[N])
